simulink model "ideal_source_Motor_DVS_newest_param"  (R2025a)
settings: Solver=daessc  StartTime=0.0  StopTime=2  MaxStep=1e-7  RelTol=1e-3
model workspace (MAT data in the model file):
  FocDiscrTime = 0.0001
  Is_max = 390
  Ld = 0.0002
  Lq = 0.0002
  PolePairs = 13
  Psi = 0.07437
  Rs = 0.06
  compensate_pwm = 0
  piBandwidth = 5000
libraries: fl_lib x18, nesl_utility x15, mcbeeMathTransformLib x7, spsMeanLib x5, slpidlib x5, simulink x2, ee_lib x1, simulink_extras x1
(part 2 of 2)

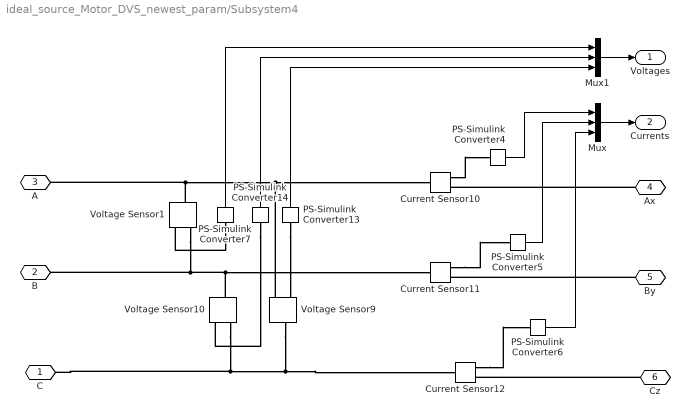
== system ideal_source_Motor_DVS_newest_param/Subsystem4 ==
  Current Sensor10 : fl_lib/Electrical/Electrical Sensors/Current Sensor
  Current Sensor11 : fl_lib/Electrical/Electrical Sensors/Current Sensor
  Current Sensor12 : fl_lib/Electrical/Electrical Sensors/Current Sensor
  Mux : Mux  Inputs=3
  Mux1 : Mux  Inputs=3
  PS-Simulink Converter{4..7,13..14} (6 alike) : nesl_utility/PS-Simulink Converter  PhysicalDomain=network_engine_domain  SubClassName=ps_output  LeftPortType=input  RightPortType=output  PseudoPeriodic=off  Frequencies=[]  VectorFormat=inherit  Unit=inherit  AffineConversion=off
  Voltage Sensor1 : fl_lib/Electrical/Electrical Sensors/Voltage Sensor
  Voltage Sensor10 : fl_lib/Electrical/Electrical Sensors/Voltage Sensor
  Voltage Sensor9 : fl_lib/Electrical/Electrical Sensors/Voltage Sensor
  C : PMIOPort  Side=Left
  B : PMIOPort  Port=2  Side=Left
  A : PMIOPort  Port=3  Side=Left
  Ax : PMIOPort  Port=4  Side=Right
  By : PMIOPort  Port=5  Side=Right
  Cz : PMIOPort  Port=6  Side=Right
  Voltages : Outport
  Currents : Outport  Port=2
  wires:
  PS-Simulink Converter5/1 -> Mux/2
  PS-Simulink Converter6/1 -> Mux/3
  PS-Simulink Converter13/1 -> Mux1/3
  PS-Simulink Converter4/1 -> Mux/1
  PS-Simulink Converter14/1 -> Mux1/2
  PS-Simulink Converter7/1 -> Mux1/1
  Mux/1 -> Currents/1
  Mux1/1 -> Voltages/1
  connections:
  Ax/RConn1 -- Current Sensor10/RConn2
  PS-Simulink Converter13/LConn1 -- Voltage Sensor9/RConn1
  Current Sensor10/RConn1 -- PS-Simulink Converter4/LConn1
  Cz/RConn1 -- Current Sensor12/RConn2
  Current Sensor11/RConn1 -- PS-Simulink Converter5/LConn1
  Voltage Sensor10/RConn2 -- C/RConn1 -- Current Sensor12/LConn1 -- Voltage Sensor9/LConn1
  Voltage Sensor1/LConn1 -- A/RConn1 -- Current Sensor10/LConn1 -- Voltage Sensor9/RConn2
  Current Sensor12/RConn1 -- PS-Simulink Converter6/LConn1
  Voltage Sensor10/LConn1 -- B/RConn1 -- Voltage Sensor1/RConn2 -- Current Sensor11/LConn1
  PS-Simulink Converter14/LConn1 -- Voltage Sensor10/RConn1
  PS-Simulink Converter7/LConn1 -- Voltage Sensor1/RConn1
  By/RConn1 -- Current Sensor11/RConn2

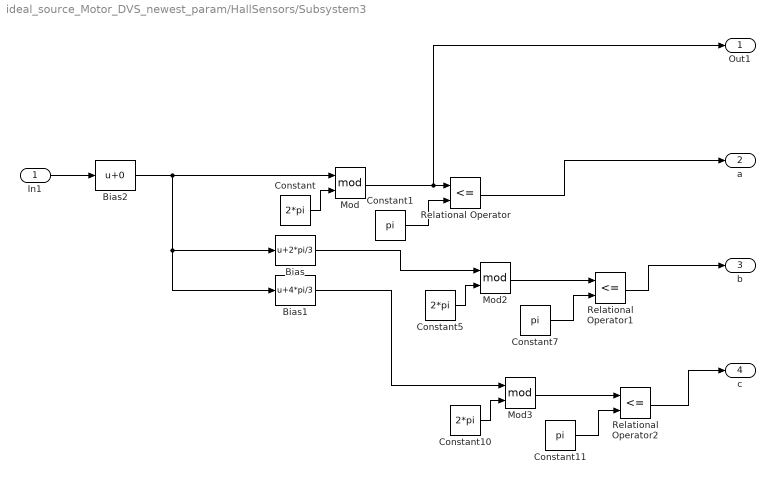
== system ideal_source_Motor_DVS_newest_param/HallSensors/Subsystem3 ==
  In1 : Inport
  Bias : Bias  Bias=2*pi/3  SaturateOnIntegerOverflow=off
  Bias1 : Bias  Bias=4*pi/3  SaturateOnIntegerOverflow=off
  Bias2 : Bias  SaturateOnIntegerOverflow=off
  Constant : Constant  Value=2*pi
  Constant1 : Constant  Value=pi
  Constant10 : Constant  Value=2*pi
  Constant11 : Constant  Value=pi
  Constant5 : Constant  Value=2*pi
  Constant7 : Constant  Value=pi
  Mod : Math  Operator=mod
  Mod2 : Math  Operator=mod
  Mod3 : Math  Operator=mod
  Relational Operator : RelationalOperator  Operator=<=  OutDataTypeStr=boolean  RndMeth=Simplest  InputSameDT=off
  Relational Operator1 : RelationalOperator  Operator=<=  OutDataTypeStr=boolean  RndMeth=Simplest  InputSameDT=off
  Relational Operator2 : RelationalOperator  Operator=<=  OutDataTypeStr=boolean  RndMeth=Simplest  InputSameDT=off
  Out1 : Outport
  "a " : Outport  Port=2
  b : Outport  Port=3
  c : Outport  Port=4
  wires:
  Bias2/1 -> Mod/1, Bias/1, Bias1/1
  In1/1 -> Bias2/1
  Mod3/1 -> Relational Operator2/1
  Relational Operator/1 -> "a "/1
  Constant1/1 -> Relational Operator/2
  Constant/1 -> Mod/2
  Constant10/1 -> Mod3/2
  Constant11/1 -> Relational Operator2/2
  Mod2/1 -> Relational Operator1/1
  Bias1/1 -> Mod3/1
  Mod/1 -> Relational Operator/1, Out1/1
  Constant7/1 -> Relational Operator1/2
  Relational Operator2/1 -> c/1
  Relational Operator1/1 -> b/1
  Constant5/1 -> Mod2/2
  Bias/1 -> Mod2/1

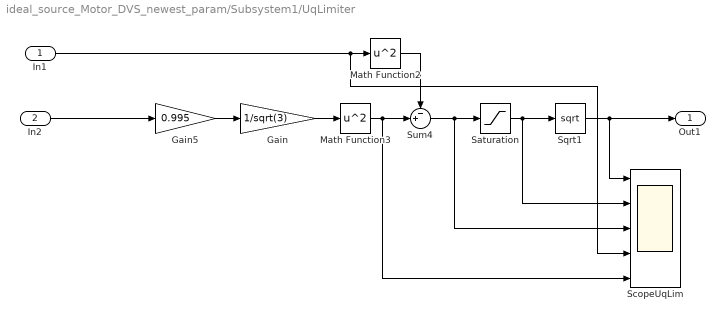
== system ideal_source_Motor_DVS_newest_param/Subsystem1/UqLimiter ==
  In1 : Inport
  In2 : Inport  Port=2
  Gain : Gain  Gain=1/sqrt(3)
  Gain5 : Gain  Gain=0.995
  Math Function2 : Math  Operator=square
  Math Function3 : Math  Operator=square
  Saturation : Saturate  UpperLimit=inf  LowerLimit=0.001
  ScopeUqLim : Scope  NumInputPorts=5
      settings: ActiveDisplayYMinimum=149.70176366248859  ActiveDisplayYMaximum=275.51811800976793  DataLoggingVariableName=ScopeData5
  Sqrt1 : Sqrt
  Sum4 : Sum  Inputs=-+|
  Out1 : Outport
  wires:
  Saturation/1 -> ScopeUqLim/2, Sqrt1/1
  Math Function3/1 -> ScopeUqLim/5, Sum4/2
  Gain/1 -> Math Function3/1
  Gain5/1 -> Gain/1
  In2/1 -> Gain5/1
  Math Function2/1 -> Sum4/1
  Sum4/1 -> ScopeUqLim/3, Saturation/1
  Sqrt1/1 -> ScopeUqLim/1, Out1/1
  In1/1 -> ScopeUqLim/4, Math Function2/1

== matlab function ideal_source_Motor_DVS_newest_param/HallSensors/MATLAB Function ==
  data: a input; ag output; b input; c input; s output
function [ag,s]= fcn(a,b,c)

dt = 1/20000;
persistent Speed;
if isempty(Speed)
    Speed = 0;
end

persistent Speed_flt;
if isempty(Speed_flt)
    Speed_flt = 0;
end


persistent cnt
if isempty(cnt)
    cnt = 0;
end

persistent com_cnt
if isempty(com_cnt)
    com_cnt = 0;
end


y = a + b * 2 + c *4;
if y == 3
    ar = pi/6;
elseif y == 1
    ar = 3*pi/6;
elseif y == 5
    ar = 5*pi/6;
elseif y == 4
    ar = 7*pi/6;
elseif y == 6
    ar = 9*pi/6;
elseif y == 2
    ar = 11*pi/6;
else 
    ar = 0;
end

ar = ar-pi/6;

persistent Angle;
if isempty(Angle)
    Angle = ar;
end

if ar ~= Angle
    f = ar - Angle;
    if f<0 
        f = f + 2*pi;
    end
    Speed_new = f/dt / (cnt+1);
    if abs(Speed_new - Speed) <  max(abs(Speed*0.5),500)
        Speed = Speed_new;
    end
    cnt = 0; 
else 
    cnt = cnt + 1;
end

%if Speed > 10000
%    Speed = 0;
%end



alfa = 0.0125;

Speed_flt = Speed_flt + alfa * (Speed - Speed_flt);

Angle = ar;







if Speed_flt < 500
    ag = ar;
else 
    ag = ar + Speed_flt*dt*(cnt +1);
end

while ag > 2*pi
    ag = ag - 2*pi;
end

s = Speed_flt;
end

== matlab function ideal_source_Motor_DVS_newest_param/SVPWM1 ==
  data: vRef input; vAngle input; VDC input; Currents input; Tat output; Tbt output; Tct output; vRefwork output; compensate_pwm parameter
function [Tat, Tbt, Tct,vRefwork] = fcn(vRef,vAngle, VDC, Currents, compensate_pwm)
%function Ts   = fcn(vrefa,vphase,VDC,IA,IB)
%время ШИМ периода
timeStamp=50e-6;
deadTime=0.0; % in us
compensate_dt = 0;
%compensate_pwm = 1;

persistent Ta_old;
persistent Tb_old;
persistent Tc_old;

if(isempty(Ta_old)||isempty(Tb_old)||isempty(Tc_old))
    Ta_old = 0.5;
    Tb_old = 0.5;
    Tc_old = 0.5;
end

persistent interruptCnt
if (isempty(interruptCnt))
    interruptCnt = true;
end


%алгоритм формирования векторной ШИМ  мертвым веменем dead [мкс]

dead_time=deadTime/(timeStamp*1e6);


if (interruptCnt)
    if (vAngle < 0)
        a = vAngle + 2*pi;
    else
        a=vAngle;
    end

    vOtn = sqrt(3) * vRef / VDC;
    if (vOtn > 0.995)
        vOtn = 0.995;
    end



    if a>=0 && a<pi/3 
        n=1;
    elseif  a>=pi/3 && a<2*pi/3 
        n=2;
    elseif  a>=2*pi/3 && a<pi 
        n=3;
    elseif  a>=pi && a<4*pi/3 
        n=4;
    elseif  a>=4*pi/3 && a<5*pi/3 
        n=5;
    else n=6;

    end

    a_cor=a-(n-1)*pi/3;

    T1 = vOtn * sin(pi/3 - a_cor);
    T2 = vOtn * sin(a_cor);
    T0=1-T1-T2;

    Ta=0; 
    Tb=0; 
    Tc=0;

    switch n
        case 1
            Ta = T1 + T2 + T0/2;
            Tb = T2 + T0/2;
            Tc = T0/2;
       
        case 2
            Ta = T1 + T0/2;
            Tb = T1 + T2 + T0/2;
            Tc = T0/2;       
        
        case 3
            Ta = T0/2;
            Tb = T1 + T2 + T0/2;
            Tc = T2 + T0/2;    
        
        case 4
            Ta = T0/2;
            Tb = T1 + T0/2;
            Tc = T1 + T2 + T0/2;   
       
        case 5
            Ta = T2 + T0/2;
            Tb = T0/2;
            Tc = T1 + T2 + T0/2;     
        
        case 6
            Ta = T1 + T2 + T0/2;
            Tb = T0/2;
            Tc = T1 + T0/2;    
        
    end

    if(compensate_pwm == 1)
        Tat = 2*Ta - Ta_old;
        Tbt = 2*Tb - Tb_old;
        Tct = 2*Tc - Tc_old;
    
    else
        Tat = Ta;
        Tbt = Tb;
        Tct = Tc;
    end

    if (Tat > 0.995)
        Tat = 0.995;
    elseif (Tat < 0.005)
        Tat = 0.005;
    end

    if (Tbt > 0.995)
        Tbt = 0.995;
    elseif (Tbt < 0.005)
        Tbt = 0.005;
    end

    if (Tct > 0.995)
        Tct = 0.995;
    elseif (Tct < 0.005)
        Tct = 0.005;
    end



    Ta_old = Ta;
    Tb_old = Tb;
    Tc_old = Tc;

else %interruptCnt
    Tat = Ta_old;
    Tbt = Tb_old;
    Tct = Tc_old;
end

        


if compensate_dt == 1
    if (Currents(1) > 0) 
        Tat = Tat - dead_time/2;
    else
        Tat = Tat + dead_time/2;
         
    end

    if (Currents(2) > 0) 
        Tbt = Tbt - dead_time/2;
    else
        Tbt = Tbt + dead_time/2;
    end

    if (-(Currents(1)+Currents(2)) > 0) 
        Tct = Tct - dead_time/2;
    else
        Tct = Tct + dead_time/2;
    end
end

interruptCnt = ~interruptCnt;
vRefwork = vRef;
return;
